simulink model "Wind_Testrig"  (R2025a)
settings: Solver=ode23t  StartTime=0.0  StopTime=400  RelTol=1e-5  EnableMultiTasking=on
PostLoadFcn:
  | warning off Simulink:blocks:MatchingGotoNotFound
  | warning off Simulink:blocks:MatchingFromNotFound
  | warning off Simulink:Engine:UsingDefaultMaxStepSize
undefined symbols (not defined in the file): Actuator_Lookup, radps2rpm, sigbuilder_block
libraries: Wind_Lib x4, sm_lib x3, Pitch_System_Lib x3, Blades_Lib x1, Pitch_Controller_Lib x1, Hub_Axis_Lib x1, nesl_utility x1
Description:
  | Copyright 2009-2025 The MathWorks, Inc. MathWorks, Inc.
settings Model: Creator=smiller  LastModifiedBy=smiller
settings SolverCC: AlgebraicLoopSolver=TrustRegion
settings DataIOCC: LimitDataPoints=on  SaveFormat=Array  ReturnWorkspaceOutputs=off
settings OptimizationCC: ReuseModelBlockBuffer=off  ExpressionDepthLimit=2147483647.0  LifeSpan=inf
settings DebuggingCC: UnderspecifiedInitializationDetection=Classic  MergeDetectMultiDrivingBlocksExec=none  SolverPrmCheckMsg=warning  FcnCallInpInsideContextMsg=warning  UnconnectedInputMsg=warning  UnconnectedOutputMsg=warning  UnconnectedLineMsg=warning  AllowSymbolicDim=off  StateNameClashWarn=warning  PregeneratedLibrarySubsystemCodeDiagnostic=none  SFUnexpectedBacktrackingDiag=warning  SFNoUnconditionalDefaultTransitionDiag=warning  SFExecutionAtInitializationDiag=none  ArithmeticOperatorsInVariantConditions=warning
settings HardwareCC: ProdBitPerPointer=32.0  ProdBitPerSizeT=32.0  ProdBitPerPtrDiffT=32.0  ProdLargestAtomicFloat=None  ProdIntDivRoundTo=Undefined  ProdEndianess=Unspecified  ProdWordSize=32.0  ProdHWDeviceType=32-bit Generic
settings ModelReferenceCC: EnableRefExpFcnMdlSchedulingChecks=on  PropagateSignalLabelsOutOfModel=off
settings SFSimCC: SimUseLocalCustomCode=off  SimParseCustomCode=off  CustomCodeUndefinedFunction=UseInterfaceOnly
settings RTWCC: RTWUseLocalCustomCode=off  GPUComputeCapability=3.5  DLArmComputeVersion=19.05
settings CodeAppCC: StateflowObjectComments=on
settings GRTTargetCC: TargetLangStandard=C89/C90 (ANSI)  CombineOutputUpdateFcns=off  GRTInterface=on
settings ConfigComp: CovMetricSettings=dw  CovSaveCumulativeToWorkspaceVar=on  CovSaveSingleToWorkspaceVar=on  CovExternalEMLEnable=off  CovSFcnEnable=off
settings SimscapeCC: SimscapeNormalizeSystem=off  SimscapeNominalValues="[{\"value\":\"10\",\"unit\":\"V\"},{\"value\":\"1\",\"unit\":\"A\"},{\"value\":\"10\",\"unit\":\"N*m\"},{\"value\":\"10\",\"unit\":\"bar\"},{\"value\":\"100\",\"unit\":\"kJ/kg\"},{\"value\":\"1\",\"unit\":\"kW\"},{\"value\":\"300\",\"unit\":\"K\"},{\"value\":\"100\",\"unit\":\"cm^3/s\"},{\"value\":\"1\",\"unit\":\"kN\"},{\"value\":\"1\",\"unit\":\"g/cm^3\"},{\"value\":\"1\",\"unit\":\"l\"},{\"value\":\"1\",\"unit\":\"cm^2\"},{\"value\":\"60\",\"unit\":\"Hz\"}]"
settings ConfigurationSet: Description=SimMechanics 2G
settings ExplorerConfigSet: InternalSimMechanicsExplorerSettings="<ExplorerConfiguration><canonicalview>default</canonicalview><TilePanel><TileInfo><Tiles Columns=\"1\" Count=\"1\" Rows=\"1\"><Column Left=\"2\" Weight=\"1\"/><Column Left=\"651\"/><Row Top=\"2\" Weight=\"1\"/><Row Top=\"510\"/><Tile Height=\"1\" Width=\"1\" X=\"0\" Y=\"0\"/></Tiles></TileInfo><SceneInfo><SceneViewer><BGColor><R>0.80000001192092896</R><G>1</G><B>1</B></BGColor><Camera><Position><X>-18.34444732617348</X><Y>-79.064377059046635</Y><Z>61.050217652840232</Z></Position><Center><X>-9.635435577615457</X><Y>1.1439116155005564</Y><Z>1.7946145717997837</Z></Center><Up><X>-0.063772345088641574</X><Y>0.59746516561897667</Y><Z>0.79935502992962004</Z></Up><Left>-34.087521171569826</Left><Right>34.087521171569826</Right><Bottom>-3.1111695885658266</Bottom><Top>3.1111695885658266</Top></Camera></SceneViewer></SceneInfo></TilePanel></ExplorerConfiguration>"

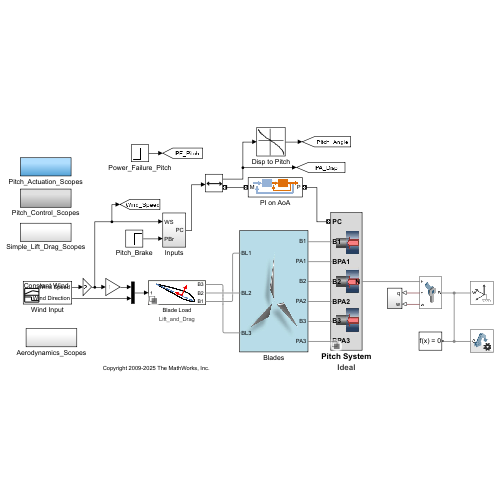
[thumbnail: Simulink's stored preview of the top-level diagram]
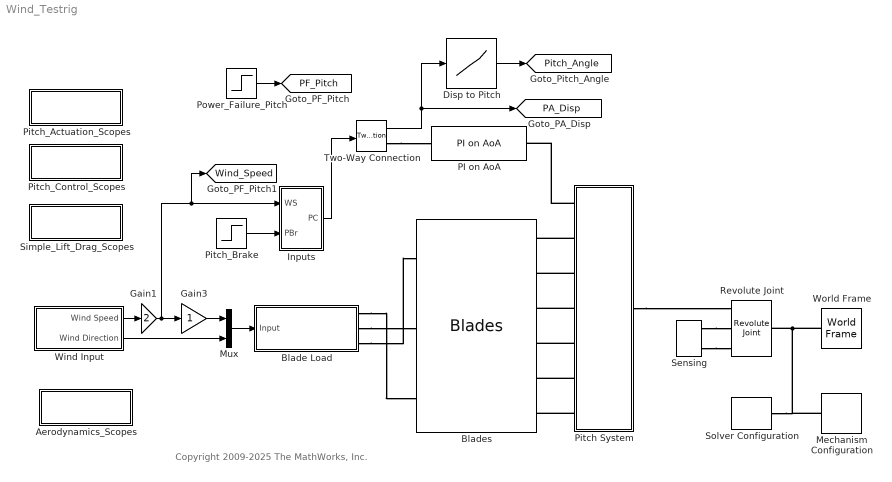
== system Wind_Testrig ==
  note: Copyright 2009-2025 The MathWorks, Inc.
  Aerodynamics_Scopes : Subsystem  AncestorBlock=Wind_Lib/Simple_Lift_Drag_Scopes
      settings: LibrarySourceBlock=Wind_Lib/Simple_Lift_Drag_Scopes
  Blade Load : Subsystem  Variant=on  VariantControlMode=label  LabelModeActiveChoice=Lift_and_Drag
      settings: AttributesFormatString=%<ActiveVariant>
      mask Display:
      | blk = wind_turbine_activeVariantBlock(gcb);
      | eval(get_param(blk, 'MaskDisplay'));
  Blades : Blades_Lib/Blades  SystemSampleTime=-1  VariantActivationTime=update diagram  EmptyChoice=off  PassThrough=off  PassThroughVariantControl=(default)  EmptyChoiceVariantControl=(default)  AllowFlexibleInterface=on  Latency=0  AutoFrameSizeCalculation=off
  Disp to Pitch : Lookup  InputValues=Actuator_Lookup.extension  Table=Actuator_Lookup.angle  SaturateOnIntegerOverflow=off
  Gain1 : Gain  Gain=2
  Gain3 : Gain
  Inputs : Subsystem
  Mechanism Configuration : sm_lib/Utilities/Mechanism Configuration  UniformGravity=Constant  GravityVector=[0 0 -9.81]  GravityVectorUnits=m/s^2  LinearizationDelta=0.001  JointModeTransitionNonlinearIterations=2
  Mux : Mux  Inputs=2
  PI on AoA : Pitch_Controller_Lib/PI on AoA  SystemSampleTime=-1  VariantActivationTime=update diagram  EmptyChoice=off  PassThrough=off  PassThroughVariantControl=(default)  EmptyChoiceVariantControl=(default)  AllowFlexibleInterface=on  Latency=0  AutoFrameSizeCalculation=off
  Pitch System : Subsystem  Tag=CustomStyle  Variant=on  VariantControlMode=label  LabelModeActiveChoice=Ideal
      settings: AttributesFormatString=%<ActiveVariant>
      mask Display:
      | blk = wind_turbine_activeVariantBlock(gcb);
      | eval(get_param(blk, 'MaskDisplay'));
  Pitch_Actuation_Scopes : Subsystem
  Pitch_Brake : Step  After=0  SampleTime=0
  Pitch_Control_Scopes : Subsystem
  Power_Failure_Pitch : Step  Time=5  Before=24  After=24  SampleTime=0
  Revolute Joint : sm_lib/Joints/Revolute Joint  JointMode=Normal  CompositeWrenchDir=FollowerOnBase  CompositeWrenchFrame=BaseFrame  SenseConstraintForce=off  SenseConstraintTorque=off  SenseTotalForce=off  SenseTotalTorque=off  PositionTargetSpecify=on  PositionTargetPriority=High  PositionTargetValue=0  PositionTargetValueUnits=deg  VelocityTargetSpecify=off  VelocityTargetPriority=High  VelocityTargetValue=0  VelocityTargetValueUnits=deg/s  EquilibriumPosition=0  EquilibriumPositionUnits=deg  SpringStiffness=0  SpringStiffnessUnits=N*m/deg  DampingCoefficient=0  DampingCoefficientUnits=N*m/(deg/s)  LowerLimitSpecify=off  LowerLimitBound=-90  LowerLimitBoundUnits=deg  LowerLimitStiffness=1e4  LowerLimitStiffnessUnits=N*m/deg  LowerLimitDamping=10  LowerLimitDampingUnits=N*m/(deg/s)  LowerLimitTransitionRegionWidth=0.1  LowerLimitTransitionRegionWidthUnits=deg  UpperLimitSpecify=off  UpperLimitBound=90  UpperLimitBoundUnits=deg  UpperLimitStiffness=1e4  UpperLimitStiffnessUnits=N*m/deg  UpperLimitDamping=10  UpperLimitDampingUnits=N*m/(deg/s)  UpperLimitTransitionRegionWidth=0.1  UpperLimitTransitionRegionWidthUnits=deg  TorqueActuationMode=NoTorque  MotionActuationMode=ComputedMotion  SensePosition=on  SenseVelocity=on  SenseAcceleration=off  SenseTorqueForce=off  SenseLowerLimitTorqueForce=off  SenseUpperLimitTorqueForce=off
  Sensing : Hub_Axis_Lib/Rotate/Sensing  SystemSampleTime=-1  VariantActivationTime=update diagram  EmptyChoice=off  PassThrough=off  PassThroughVariantControl=(default)  EmptyChoiceVariantControl=(default)  AllowFlexibleInterface=on  Latency=0  AutoFrameSizeCalculation=off
  Simple_Lift_Drag_Scopes : Subsystem  AncestorBlock=Wind_Lib/Simple_Lift_Drag_Scopes
      settings: LibrarySourceBlock=Wind_Lib/Simple_Lift_Drag_Scopes
  Solver Configuration : nesl_utility/Solver Configuration  PhysicalDomain=network_engine_domain  SubClassName=solver  LeftPortType=input  RightPortType=generic  Tones=[]  Harmonics=[]  SimulateNoise=off  Profile=off  UseLocalSampling=off  EnableSwitchedLinearOptims=on  FrequencyDomain=off  UseCCode=off  RelTol=0.001  AbsTol=1e-06  MinStep=1e-09  ToWorkspace=off  RevertToSquareIcSolve=off  NumHomotopyIterations=100  PhasorMode=off  PhasorModeNumHarmonics=1  ConsistencySolver=NEWTON_FTOL  IndexReductionMethod=DerivativeReplacement  DoDC=off  ResidualTolerance=1e-9  ConsistencyTolSource=GLOBAL  ConsistencyAbsTol=0.001  ConsistencyRelTol=0.001  ConsistencyTolFactor=0.001  UseLocalSolver=off  LocalSolverChoice=NE_BACKWARD_EULER_ADVANCER  ResolveIndetEquations=on  FunctionEvalNumThread=1  LocalSolverSampleTime=.001  DoFixedCost=off  MaxNonlinIter=3  MaxModeIter=2  ComputeImpulses=off  ImpulseIterations=2  LinearAlgebra=Sparse  LinearAlgebraNumThread=0  EquationFormulation=NE_TIME_EF  DelaysMemoryBudget=1024  AutomaticFiltering=on  FilteringTimeConstant=0.001  PartitionStorageMethod=AS_NEEDED  PartitionMemoryBudget=1024  PartitionMethod=FAST  MultibodyUseLocalSolver=off  MultibodyLocalSolverChoice=ODE1  MultibodyLocalSolverSampleTime=0.001
  Two-Way Connection : TwoWayConnection
  Wind Input : Subsystem  Tag=STV Subsys  LoadFcn=sigbuilder_block('load');  StartFcn=sigbuilder_block('start');  StopFcn=sigbuilder_block('stop');  ClipboardFcn=sigbuilder_block('clipboard');  mask(Sigbuilder block){tuvar=[0:10]}
      mask help: Sigbuilder GUI
      mask init:
      | if ~strcmp(get_param(bdroot(gcbh),'SimulationStatus'),'stopped') tuvar = sigbuilder_block('maskInit'); end
      settings: CopyFcn=sigbuilder_block('copy');  DeleteFcn=sigbuilder_block('delete');  ModelCloseFcn=sigbuilder_block('modelClose');  PreSaveFcn=sigbuilder_block('preSave');  PauseFcn=sigbuilder_block('pause')  ContinueFcn=sigbuilder_block('continue')  NameChangeFcn=sigbuilder_block('namechange');  OpenFcn=sigbuilder_block('open',[33 180 762 399.75 ]);  CloseFcn=sigbuilder_block('close');
      mask Display: plot(0, 0, 100, 100,[2, 2, 32, 32, 2], [68, 8, 8, 68, 68],[32, 2], [38, 38], [32, 19, 2],[53, 60, 44], [32, 17, 17, 2],[16, 16, 31, 31]);txt = getActiveGroup(gcbh);text(2, 100, txt,'verticalAlignment', 'top');
  World Frame : sm_lib/Frames and Transforms/World Frame
  tag scope: PA_Disp=global, PF_Pitch=global, Pitch_Angle=global, Wind_Speed=global
  wires:
  Disp to Pitch/1 -> [Pitch_Angle]
  Two-Way Connection/1 -> [PA_Disp], Disp to Pitch/1
  Power_Failure_Pitch/1 -> [PF_Pitch]
  Wind Input/1(Wind Speed) -> Gain1/1
  Wind Input/2(Wind Direction) -> Mux/2
  Mux/1 -> Blade Load/1(Input)
  Pitch_Brake/1 -> Inputs/2(PBr)
  Inputs/1(PC) -> Two-Way Connection/1
  Gain3/1 -> Mux/1
  Gain1/1 -> Gain3/1, Inputs/1(WS), [Wind_Speed]
  connections:
  Pitch System/LConn2 -- Blades/LConn1
  Pitch System/LConn6 -- Blades/LConn5
  Pitch System/LConn4 -- Blades/LConn3
  Pitch System/LConn3 -- Blades/LConn2
  Two-Way Connection/RConn1 -- PI on AoA/LConn1
  Pitch System/LConn1 -- PI on AoA/RConn1
  Pitch System/LConn5 -- Blades/LConn4
  Pitch System/LConn7 -- Blades/LConn6
  Blade Load/RConn1 -- Blades/RConn3
  Blade Load/RConn2 -- Blades/RConn2
  Sensing/LConn1 -- Revolute Joint/RConn2
  Sensing/LConn2 -- Revolute Joint/RConn3
  Pitch System/RConn1 -- Revolute Joint/RConn1
  World Frame/RConn1 -- Mechanism Configuration/RConn1 -- Solver Configuration/RConn1 -- Revolute Joint/LConn1
  Blade Load/RConn3 -- Blades/RConn1

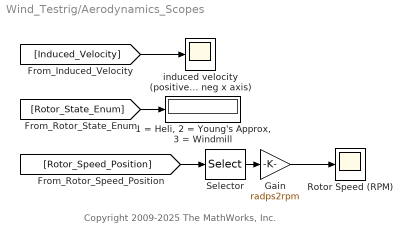
== system Wind_Testrig/Aerodynamics_Scopes ==
  note: Copyright 2009-2025 The MathWorks, Inc.
  "1 = Heli, 2 = Young's Approx, 3 = Windmill" : Display
  Gain : Gain  Gain=radps2rpm
  Rotor Speed (RPM) : Scope
      settings: TimeSpan=80  ActiveDisplayYMinimum=0  ActiveDisplayYMaximum=12  DataLoggingVariableName=ScopeData11
  Selector : Selector  InputPortWidth=2  IndexOptions=Index vector (dialog)  Indices=[2]  OutputSizes=1
  induced velocity (positive in neg x axis) : Scope
      settings: TimeSpan=100  ActiveDisplayYMinimum=-8  ActiveDisplayYMaximum=4  DataLoggingVariableName=ScopeData12
  wires:
  [Rotor_State_Enum] -> "1 = Heli, 2 = Young's Approx, 3 = Windmill"/1
  [Induced_Velocity] -> induced velocity (positive in neg x axis)/1
  [Rotor_Speed_Position] -> Selector/1
  Selector/1 -> Gain/1
  Gain/1 -> Rotor Speed (RPM)/1

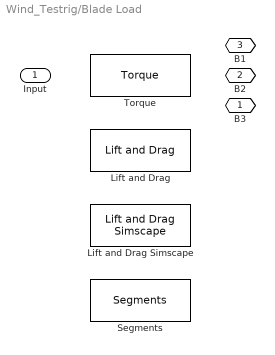
== system Wind_Testrig/Blade Load ==
  Input : Inport
  Lift and Drag : Wind_Lib/Lift and Drag  SystemSampleTime=-1  VariantControl=Lift_and_Drag  VariantActivationTime=update diagram  EmptyChoice=off  PassThrough=off  PassThroughVariantControl=(default)  EmptyChoiceVariantControl=(default)  AllowFlexibleInterface=on  Latency=0  AutoFrameSizeCalculation=off
  Lift and Drag Simscape : Wind_Lib/Lift and Drag Simscape  SystemSampleTime=-1  VariantControl=Lift_and_Drag_Simscape  VariantActivationTime=update diagram  EmptyChoice=off  PassThrough=off  PassThroughVariantControl=(default)  EmptyChoiceVariantControl=(default)  AllowFlexibleInterface=on  Latency=0  AutoFrameSizeCalculation=off
  Segments : Wind_Lib/Segments  SystemSampleTime=-1  VariantControl=Segments  VariantActivationTime=update diagram  EmptyChoice=off  PassThrough=off  PassThroughVariantControl=(default)  EmptyChoiceVariantControl=(default)  AllowFlexibleInterface=on  Latency=0  AutoFrameSizeCalculation=off
  Torque : Wind_Lib/Torque  SystemSampleTime=-1  VariantControl=Torque  VariantActivationTime=update diagram  EmptyChoice=off  PassThrough=off  PassThroughVariantControl=(default)  EmptyChoiceVariantControl=(default)  AllowFlexibleInterface=on  Latency=0  AutoFrameSizeCalculation=off
  B3 : PMIOPort  Side=Right
  B2 : PMIOPort  Port=2  Side=Right
  B1 : PMIOPort  Port=3  Side=Right

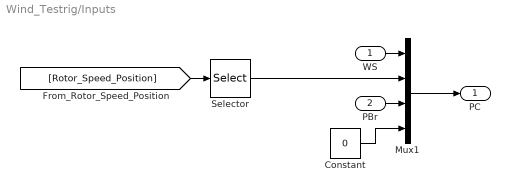
== system Wind_Testrig/Inputs ==
  WS : Inport
  PBr : Inport  Port=2
  Constant : Constant  Value=0
  Mux1 : Mux
  Selector : Selector  InputPortWidth=2  IndexOptions=Index vector (dialog)  Indices=[2]  OutputSizes=1
  PC : Outport  VectorParamsAs1DForOutWhenUnconnected=off
  wires:
  [Rotor_Speed_Position] -> Selector/1
  Selector/1 -> Mux1/2
  WS/1 -> Mux1/1
  Mux1/1 -> PC/1
  PBr/1 -> Mux1/3
  Constant/1 -> Mux1/4

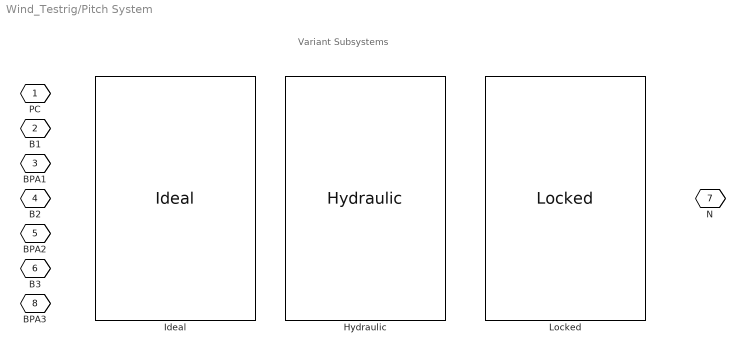
== system Wind_Testrig/Pitch System ==
  note: Variant Subsystems
  Hydraulic : Pitch_System_Lib/Hydraulic  SystemSampleTime=-1  VariantControl=Hydraulic  VariantActivationTime=update diagram  EmptyChoice=off  PassThrough=off  PassThroughVariantControl=(default)  EmptyChoiceVariantControl=(default)  AllowFlexibleInterface=on  Latency=0  AutoFrameSizeCalculation=off
  Ideal : Pitch_System_Lib/Ideal  SystemSampleTime=-1  VariantControl=Ideal  VariantActivationTime=update diagram  EmptyChoice=off  PassThrough=off  PassThroughVariantControl=(default)  EmptyChoiceVariantControl=(default)  AllowFlexibleInterface=on  Latency=0  AutoFrameSizeCalculation=off
  Locked : Pitch_System_Lib/Locked  SystemSampleTime=-1  VariantControl=Locked  VariantActivationTime=update diagram  EmptyChoice=off  PassThrough=off  PassThroughVariantControl=(default)  EmptyChoiceVariantControl=(default)  AllowFlexibleInterface=on  Latency=0  AutoFrameSizeCalculation=off
  PC : PMIOPort  Tag=PMCPort  Side=Left
  B1 : PMIOPort  Tag=PMCPort  Port=2  Side=Left
  BPA1 : PMIOPort  Tag=PMCPort  Port=3  Side=Left
  B2 : PMIOPort  Tag=PMCPort  Port=4  Side=Left
  BPA2 : PMIOPort  Tag=PMCPort  Port=5  Side=Left
  B3 : PMIOPort  Tag=PMCPort  Port=6  Side=Left
  N : PMIOPort  Tag=PMCPort  Port=7  Side=Right
  BPA3 : PMIOPort  Tag=PMCPort  Port=8  Side=Left

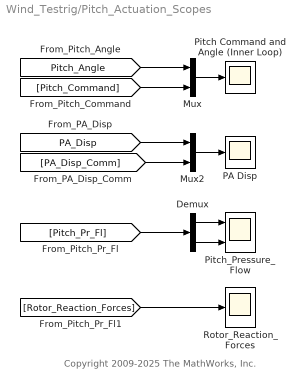
== system Wind_Testrig/Pitch_Actuation_Scopes ==
  note: Copyright 2009-2025 The MathWorks, Inc.
  Demux : Demux  Outputs=[2 1]
  Mux : Mux  Inputs=2
  Mux2 : Mux  Inputs=2
  PA Disp : Scope
      settings: TimeSpan=10  ActiveDisplayYMinimum=-1.6  ActiveDisplayYMaximum=-0.9
  Pitch Command and Angle (Inner Loop) : Scope
      settings: TimeSpan=400  ActiveDisplayYMinimum=-20  ActiveDisplayYMaximum=80
  Pitch_Pressure_Flow : Scope  NumInputPorts=2
      settings: TimeSpan=10  ActiveDisplayYMinimum=-5.0E+6  ActiveDisplayYMaximum=2.5E+7  DataLoggingVariableName=ScopeData3
  Rotor_Reaction_Forces : Scope
      settings: TimeSpan=10  ActiveDisplayYMinimum=-5.0E+6  ActiveDisplayYMaximum=2.5E+7  DataLoggingVariableName=ScopeData15
  wires:
  [Pitch_Angle] -> Mux/1
  [Pitch_Command] -> Mux/2
  Mux/1 -> Pitch Command and Angle (Inner Loop)/1
  [PA_Disp] -> Mux2/1
  Mux2/1 -> PA Disp/1
  [PA_Disp_Comm] -> Mux2/2
  [Pitch_Pr_Fl] -> Demux/1
  Demux/1 -> Pitch_Pressure_Flow/1
  Demux/2 -> Pitch_Pressure_Flow/2
  [Rotor_Reaction_Forces] -> Rotor_Reaction_Forces/1

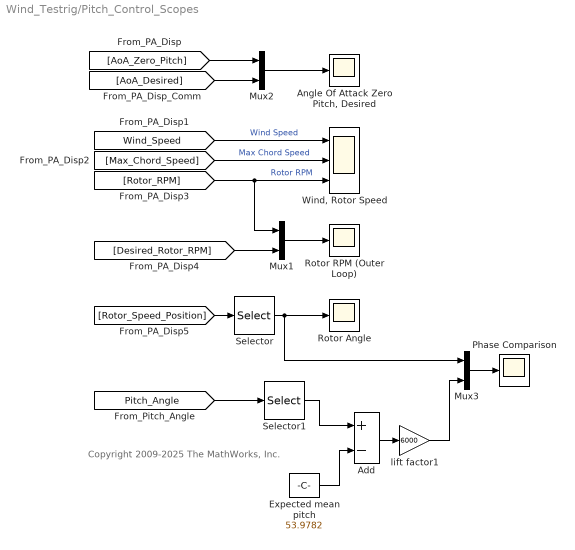
== system Wind_Testrig/Pitch_Control_Scopes ==
  note: Copyright 2009-2025 The MathWorks, Inc.
  Add : Sum  Inputs=+-
  "Angle Of Attack Zero Pitch, Desired" : Scope
      settings: TimeSpan=400  ActiveDisplayYMinimum=-40  ActiveDisplayYMaximum=100
  Expected mean pitch : Constant  Value=53.9782
  Mux1 : Mux  Inputs=2
  Mux2 : Mux  Inputs=2
  Mux3 : Mux  Inputs=2
  Phase Comparison : Scope
      settings: TimeSpan=10.02528256989888  ActiveDisplayYMinimum=-4  ActiveDisplayYMaximum=4  DataLoggingVariableName=ScopeData16
  Rotor Angle : Scope
      settings: TimeSpan=10.02528256989888  ActiveDisplayYMinimum=-4  ActiveDisplayYMaximum=4  DataLoggingVariableName=ScopeData7
  Rotor RPM (Outer Loop) : Scope
      settings: TimeSpan=400  ActiveDisplayYMaximum=20  DataLoggingVariableName=ScopeData13
  Selector : Selector  InputPortWidth=2  IndexOptions=Index vector (dialog)  Indices=[1]  OutputSizes=1
  Selector1 : Selector  InputPortWidth=3  IndexOptions=Index vector (dialog)  Indices=[1]  OutputSizes=1
  "Wind, Rotor Speed" : Scope  NumInputPorts=3
      settings: TimeSpan=600  ActiveDisplayYMinimum=5  ActiveDisplayYMaximum=15  DataLoggingVariableName=ScopeData2
  lift factor1 : Gain  Gain=6000
  wires:
  [AoA_Desired] -> Mux2/2
  Mux2/1 -> "Angle Of Attack Zero Pitch, Desired"/1
  [AoA_Zero_Pitch] -> Mux2/1
  [Wind_Speed] -> "Wind, Rotor Speed"/1  "Wind Speed"
  [Max_Chord_Speed] -> "Wind, Rotor Speed"/2  "Max Chord Speed"
  [Rotor_RPM] -> "Wind, Rotor Speed"/3, Mux1/1  "Rotor RPM"
  Mux1/1 -> Rotor RPM (Outer Loop)/1
  [Desired_Rotor_RPM] -> Mux1/2
  [Rotor_Speed_Position] -> Selector/1
  Selector/1 -> Rotor Angle/1, Mux3/1
  Mux3/1 -> Phase Comparison/1
  Expected mean pitch/1 -> Add/2
  [Pitch_Angle] -> Selector1/1
  Selector1/1 -> Add/1
  Add/1 -> lift factor1/1
  lift factor1/1 -> Mux3/2

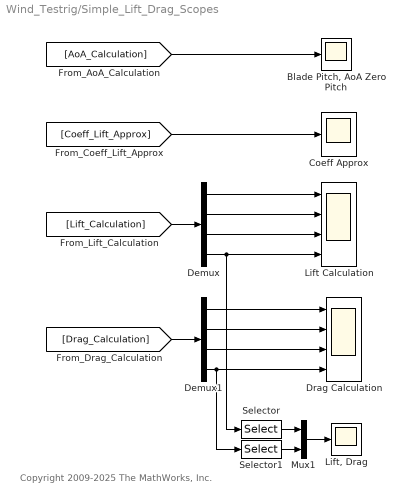
== system Wind_Testrig/Simple_Lift_Drag_Scopes ==
  note: Copyright 2009-2025 The MathWorks, Inc.
  "Blade Pitch, AoA Zero Pitch" : Scope
      settings: TimeSpan=400  ActiveDisplayYMinimum=0  ActiveDisplayYMaximum=100  DataLoggingVariableName=ScopeData3
  Coeff Approx : Scope
      settings: TimeSpan=400  ActiveDisplayYMinimum=-0.1139986551164904  ActiveDisplayYMaximum=0.01794057021302797  DataLoggingVariableName=ScopeData4
  Demux : Demux  Outputs=[1 3 3 3]
  Demux1 : Demux  Outputs=[1 3 3 3]
  Drag Calculation : Scope  NumInputPorts=4
      settings: TimeSpan=400  ActiveDisplayYMinimum=-2000  ActiveDisplayYMaximum=4000  DataLoggingVariableName=ScopeData5
  Lift Calculation : Scope  NumInputPorts=4
      settings: TimeSpan=400  ActiveDisplayYMinimum=0  ActiveDisplayYMaximum=2000  DataLoggingVariableName=ScopeData2
  "Lift, Drag" : Scope
      settings: TimeSpan=160  ActiveDisplayYMinimum=-250.43517596694389  ActiveDisplayYMaximum=408.30262213523071
  Mux1 : Mux  Inputs=2
  Selector : Selector  InputPortWidth=3  IndexOptions=Index vector (dialog)  Indices=[1]  OutputSizes=1
  Selector1 : Selector  InputPortWidth=3  IndexOptions=Index vector (dialog)  Indices=[1 3]  OutputSizes=1
  wires:
  Demux1/4 -> Drag Calculation/4, Selector1/1
  Demux1/3 -> Drag Calculation/3
  Demux1/2 -> Drag Calculation/2
  Demux1/1 -> Drag Calculation/1
  [Drag_Calculation] -> Demux1/1
  [Coeff_Lift_Approx] -> Coeff Approx/1
  Demux/4 -> Lift Calculation/4, Selector/1
  Demux/3 -> Lift Calculation/3
  Demux/2 -> Lift Calculation/2
  Demux/1 -> Lift Calculation/1
  [Lift_Calculation] -> Demux/1
  Mux1/1 -> "Lift, Drag"/1
  [AoA_Calculation] -> "Blade Pitch, AoA Zero Pitch"/1
  Selector/1 -> Mux1/1
  Selector1/1 -> Mux1/2

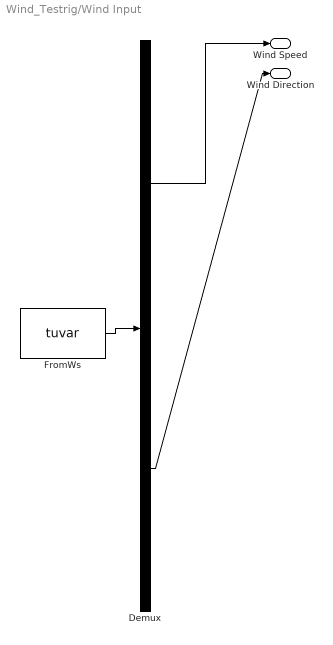
== system Wind_Testrig/Wind Input ==
  Demux : Demux  Tag=STV Demux  Outputs=2
      settings: DisplayOption=none
  FromWs : FromWorkspace  Tag=STV FromWs  VariableName=tuvar
      SigBuilderData=|
      | common.afterFinalStr = 'Extrapolate'
      | common.sampleTime = 0
      | dataSet(1).timeRange = [0 130]
      | dataSet(1).name = 'High Wind Speed'
      | dataSet(2).timeRange = [0 130]
      | dataSet(2).name = 'Constant Wind'
      | dataSet(3).timeRange = [0 130]
      | dataSet(3).name = 'Cut In'
      | sbobj.Groups(1).Name = 'High Wind Speed'
      | sbobj.Groups(1).Signals(1).Name = 'Wind Speed'
      | sbobj.Groups(1).Signals(1).XData = [0 10 10 25.1 28 91.8 100 130]
      | sbobj.Groups(1).Signals(1).YData = [10 10 9.9 9.9 5 5 8 10]
      | sbobj.Groups(1).Signals(2).Name = 'Wind Direction'
      | sbobj.Groups(1).Signals(2).XData = [0 1 1 11 11 21 21 31 31 130]
      | sbobj.Groups(1).Signals(2).YData = [0 0 4 4 0 0 -4 -4 0 0]
      | sbobj.Groups(2).Name = 'Constant Wind'
      | sbobj.Groups(2).Signals(1).Name = 'Wind Speed'
      | sbobj.Groups(2).Signals(1).XData = [0 10 130]
      | sbobj.Groups(2).Signals(1).YData = [10 10 10]
      | sbobj.Groups(2).Signals(2).Name = 'Wind Direction'
      | sbobj.Groups(2).Signals(2).XData = [0 1 1 11 11 21 21 31 31 130]
      | sbobj.Groups(2).Signals(2).YData = [0 0 4 4 0 0 -4 -4 0 0]
      | sbobj.Groups(3).Name = 'Cut In'
      | sbobj.Groups(3).Signals(1).Name = 'Wind Speed'
      | sbobj.Groups(3).Signals(1).XData = [0 25.1 28 91.8 100 121.8 130]
      | sbobj.Groups(3).Signals(1).YData = [4.5 8.7 7.85 9.65 8 10 10]
      | sbobj.Groups(3).Signals(2).Name = 'Wind Direction'
      | sbobj.Groups(3).Signals(2).XData = [0 1 1 11 11 21 21 31 31 130]
      | sbobj.Groups(3).Signals(2).YData = [0 0 4 4 0 0 -4 -4 0 0]
  Wind Speed : Outport  Tag=STV Outport  VectorParamsAs1DForOutWhenUnconnected=off
  Wind Direction : Outport  Tag=STV Outport  Port=2  VectorParamsAs1DForOutWhenUnconnected=off
  wires:
  Demux/2 -> Wind Direction/1
  Demux/1 -> Wind Speed/1
  FromWs/1 -> Demux/1
